simulink model "MassDampedSpring"  (R2026b)
settings: Solver=VariableStepAuto  StopTime=20
model workspace (MAT data in the model file):
  c = 4
  k = 15
  m = 2
settings Model: Creator=ALP  LastModifiedBy=ALP
settings DebuggingCC: AlgebraicLoopMsg=none

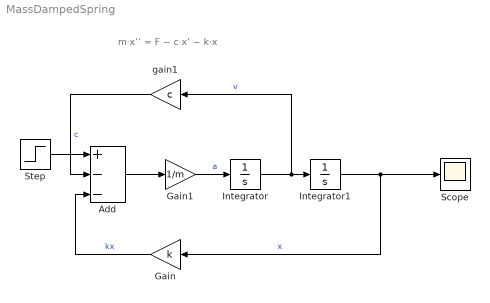
== system MassDampedSpring ==
  note: m·x’’ = F − c·x’ − k·x
  Add : Sum  Inputs=+--
  Gain : Gain  Gain=k
  Gain1 : Gain  Gain=1/m
  Integrator : Integrator
  Integrator1 : Integrator  InitialCondition=5
  Scope : Scope
      settings: ActiveDisplayYMinimum=-7.4432921678687212  ActiveDisplayYMaximum=9.6423191714754264
  Step : Step  SampleTime=0
  gain1 : Gain  Gain=c
  wires:
  Gain/1 -> Add/3  "kx"
  Add/1 -> Gain1/1
  Gain1/1 -> Integrator/1  "a"
  Integrator/1 -> gain1/1, Integrator1/1  "v"
  Integrator1/1 -> Gain/1, Scope/1  "x"
  gain1/1 -> Add/2  "c"
  Step/1 -> Add/1
